simulink model "SMO_lab10"  (R2025b)
settings: Solver=FixedStepDiscrete  StartTime=0.0  StopTime=4000  RelTol=1e-3
values from neighbouring files (symbols this model uses):
  m = 'SMO_lab10'    [lab10.m]
undefined symbols (not defined in the file or in its folder): n
settings Model: Creator=saliy_03jey6u  LastModifiedBy=saliy_03jey6u

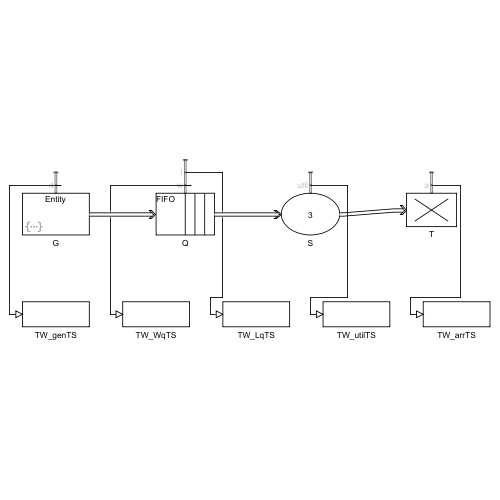
[thumbnail: Simulink's stored preview of the top-level diagram]
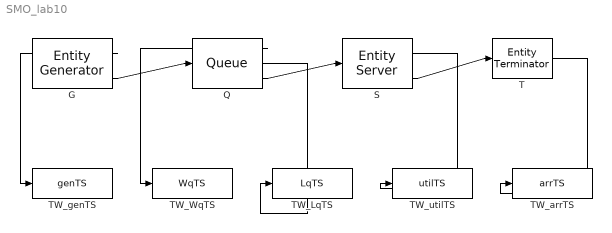
== system SMO_lab10 ==
  G : EntityGenerator  OutputPortMessageModes=n,m  TimeSource=MATLAB action  IntergenerationTimeAction=dt = -log(rand())/2.5;  GenerateAction=st = -log(rand())/1;  AttributeName=st  NumberEntitiesDeparted=on  EntityType=Structured  EntityTypeName=Entity
      settings: OutputPortMap=o0,o3
  Q : Queue  InputPortMessageModes=m  OutputPortMessageModes=n,n,m  Capacity=100  AverageWait=on  AverageQueueLength=on
      settings: OutputPortMap=o2,o3,o5
  S : EntityServer  InputPortMessageModes=m  OutputPortMessageModes=n,m  Capacity=3  ServiceTimeSource=Attribute  ServiceTimeAttributeName=st  Utilization=on
      settings: OutputPortMap=o5,o9
  T : EntityTerminator  InputPortMessageModes=m  NumberEntitiesArrived=on
      settings: OutputPortMap=o0
  TW_LqTS : ToWorkspace  VariableName=LqTS  SaveFormat=Timeseries  SampleTime=-1
  TW_WqTS : ToWorkspace  VariableName=WqTS  SaveFormat=Timeseries  SampleTime=-1
  TW_arrTS : ToWorkspace  VariableName=arrTS  SaveFormat=Timeseries  SampleTime=-1
  TW_genTS : ToWorkspace  VariableName=genTS  SaveFormat=Timeseries  SampleTime=-1
  TW_utilTS : ToWorkspace  VariableName=utilTS  SaveFormat=Timeseries  SampleTime=-1
  wires:
  G/2 -> Q/1
  Q/3 -> S/1
  S/2 -> T/1
  G/1 -> TW_genTS/1
  Q/1 -> TW_WqTS/1
  Q/2 -> TW_LqTS/1
  S/1 -> TW_utilTS/1
  T/1 -> TW_arrTS/1
